simulink model "x1_foc_transform"  (R2024b)
settings: Solver=VariableStepAuto  StartTime=0.0  StopTime=0.5  RelTol=1e-3
undefined symbols (not defined in the file or in its folder): DiscIntNeverNeededParam, Ts
libraries: spspowerguiLib x1
settings Model: Creator=disnox  LastModifiedBy=cd
settings DataIOCC: ReturnWorkspaceOutputs=off
settings DebuggingCC: ParameterPrecisionLossMsg=none
settings RTWCC: GPUComputeCapability=3.5

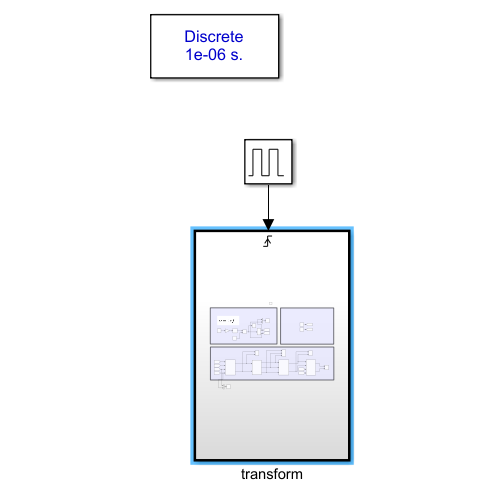
[thumbnail: Simulink's stored preview of the top-level diagram]
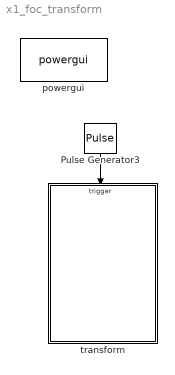
== system x1_foc_transform ==
  Pulse Generator3 : DiscretePulseGenerator  PulseType=Time based  Period=Ts  PulseWidth=50
  powergui : spspowerguiLib/powergui  SimulationMode=Discrete  SampleTime=Ts/100  frequency=60  Iterations=50  frequencyindice=0  Pbase=100e6  ErrMax=1e-4  UnitsV=kV  UnitsW=MW  buscounter=0  FunctionMessages=off  echomessages=off  EnableUseOfTLC=off  CurrentSourceSwitches=off  DisableSnubberDevices=off  DisableRonSwitches=off  DisableVfSwitches=off  DisplayEquations=off  AutomaticDiscreteSolvers=off  SolverType=Tustin/Backward Euler (TBE)  Interpol=off  ExternalGateDelay=off  methode=off  Ts=0  x0status=blocks  SPID=off  SwTol=0  HookPort=off  NonlinearTolerance=1e-4  nMaxIteration=100  ContinueOnMaxIteration=off  RestoreLinks=warning  ResistiveCurrentMeasurement=off  Frange=[0:2:500]  Ylog=off  Xlog=on  ShowGrid=off  save=off  variable=ZData  structure=0  ZoomFFT=off  StartTime=0.0  cycles=1  DisplayStyle=1  fundamental=60  FreqAxis=off  MaxFrequency=1000  frequencyindicesteady=1  RmsSteady=1  display=off
  transform : Subsystem
  wires:
  Pulse Generator3/1 -> transform/Trigger

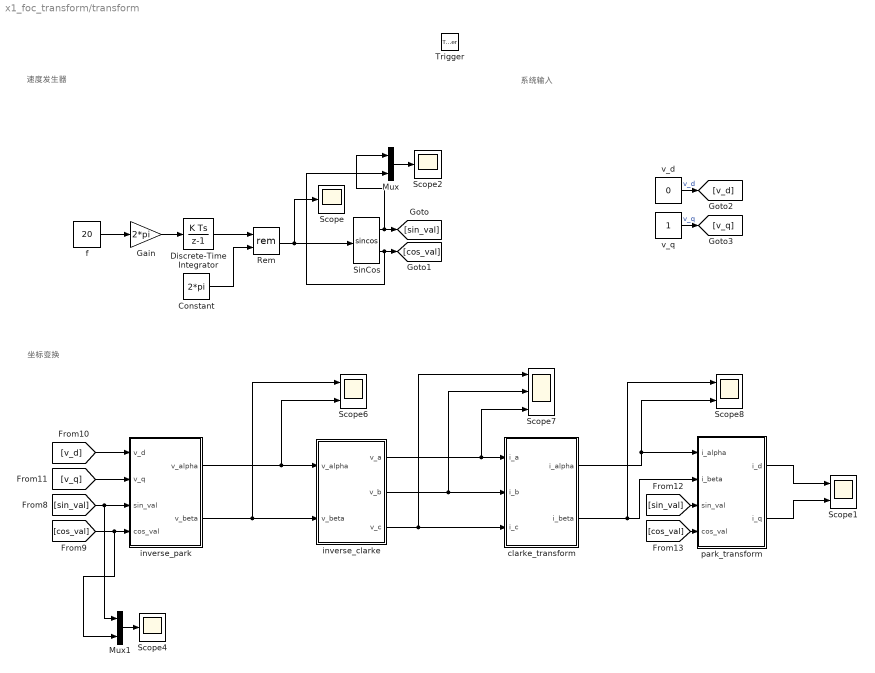
== system x1_foc_transform/transform ==
  note: 系统输入
  note: 速度发生器
  note: 坐标变换
  Trigger : TriggerPort  VariantControl=(inherit)
  Constant : Constant  Value=2*pi
  Discrete-Time Integrator : DiscreteIntegrator  SampleTime=-1  ICPrevOutput=DiscIntNeverNeededParam  ICPrevScaledInput=DiscIntNeverNeededParam
  Gain : Gain  Gain=2*pi
  Mux : Mux  Inputs=2
  Mux1 : Mux  Inputs=2
  Rem : Math  Operator=rem
  Scope : Scope
  Scope1 : Scope  NumInputPorts=2
  Scope2 : Scope
  Scope4 : Scope
  Scope6 : Scope  NumInputPorts=2
  Scope7 : Scope  NumInputPorts=3
  Scope8 : Scope  NumInputPorts=2
  SinCos : Trigonometry  Operator=sincos
  clarke_transform : Subsystem  TreatAsAtomicUnit=on
      settings: RTWSystemCode=Nonreusable function  RTWFcnNameOpts=Use subsystem name
  f : Constant  Value=20
  inverse_clarke : Subsystem  TreatAsAtomicUnit=on
      settings: RTWSystemCode=Nonreusable function  RTWFcnNameOpts=Use subsystem name
  inverse_park : Subsystem  TreatAsAtomicUnit=on
      settings: RTWSystemCode=Nonreusable function  RTWFcnNameOpts=Use subsystem name
  park_transform : Subsystem  TreatAsAtomicUnit=on
      settings: RTWSystemCode=Nonreusable function  RTWFcnNameOpts=Use subsystem name
  v_d : Constant  Value=0
  v_q : Constant
  wires:
  SinCos/1 -> Mux/1, [sin_val]
  SinCos/2 -> Mux/2, [cos_val]
  v_q/1 -> [v_q]  "v_q"
  v_d/1 -> [v_d]  "v_d"
  [cos_val] -> Mux1/2, inverse_park/4(cos_val)
  [sin_val] -> park_transform/3(sin_val)
  [v_d] -> inverse_park/1(v_d)
  [v_q] -> inverse_park/2(v_q)
  [cos_val] -> park_transform/4(cos_val)
  [sin_val] -> Mux1/1, inverse_park/3(sin_val)
  inverse_park/1(v_alpha) -> Scope6/2, inverse_clarke/1(v_alpha)
  clarke_transform/1(i_alpha) -> Scope8/2, park_transform/1(i_alpha)
  clarke_transform/2(i_beta) -> Scope8/1, park_transform/2(i_beta)
  inverse_clarke/1(v_a) -> Scope7/3, clarke_transform/1(i_a)
  inverse_clarke/3(v_c) -> clarke_transform/3(i_c), Scope7/1
  inverse_clarke/2(v_b) -> Scope7/2, clarke_transform/2(i_b)
  inverse_park/2(v_beta) -> Scope6/1, inverse_clarke/2(v_beta)
  park_transform/1(i_d) -> Scope1/1
  park_transform/2(i_q) -> Scope1/2
  Constant/1 -> Rem/2
  f/1 -> Gain/1
  Gain/1 -> Discrete-Time Integrator/1
  Discrete-Time Integrator/1 -> Rem/1
  Rem/1 -> SinCos/1, Scope/1
  Mux/1 -> Scope2/1
  Mux1/1 -> Scope4/1

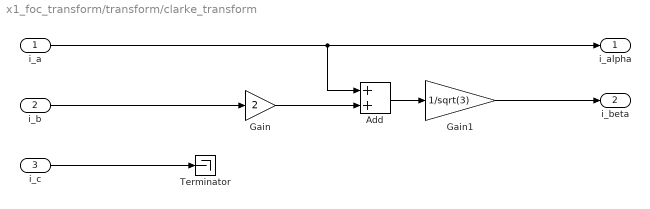
== system x1_foc_transform/transform/clarke_transform ==
  i_a : Inport
  i_b : Inport  Port=2
  i_c : Inport  Port=3
  Add : Sum
  Gain : Gain  Gain=2
  Gain1 : Gain  Gain=1/sqrt(3)
  Terminator : Terminator
  i_alpha : Outport
  i_beta : Outport  Port=2
  wires:
  i_a/1 -> Add/1, i_alpha/1
  i_b/1 -> Gain/1
  Gain/1 -> Add/2
  Add/1 -> Gain1/1
  Gain1/1 -> i_beta/1
  i_c/1 -> Terminator/1

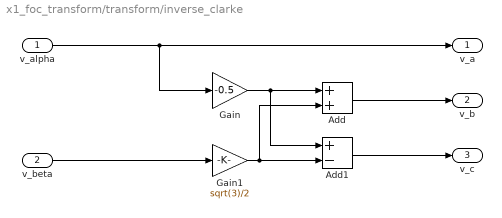
== system x1_foc_transform/transform/inverse_clarke ==
  v_alpha : Inport
  v_beta : Inport  Port=2
  Add : Sum
  Add1 : Sum  Inputs=+-
  Gain : Gain  Gain=-0.5
  Gain1 : Gain  Gain=sqrt(3)/2
  v_a : Outport
  v_b : Outport  Port=2
  v_c : Outport  Port=3
  wires:
  v_alpha/1 -> Gain/1, v_a/1
  Gain/1 -> Add1/1, Add/1
  v_beta/1 -> Gain1/1
  Gain1/1 -> Add/2, Add1/2
  Add/1 -> v_b/1
  Add1/1 -> v_c/1

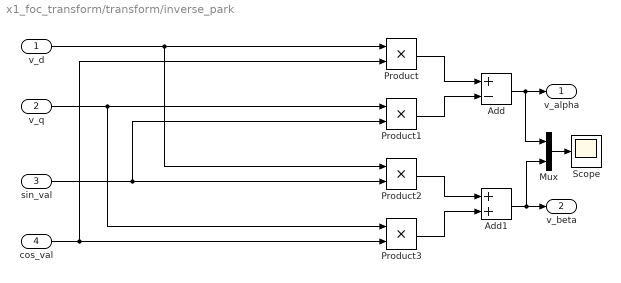
== system x1_foc_transform/transform/inverse_park ==
  v_d : Inport
  v_q : Inport  Port=2
  sin_val : Inport  Port=3
  cos_val : Inport  Port=4
  Add : Sum  Inputs=+-
  Add1 : Sum  AccumDataTypeStr=double
  Mux : Mux  Inputs=2
  Product{,1..3} (4 alike) : Product
  Scope : Scope
  v_alpha : Outport
  v_beta : Outport  Port=2
  wires:
  v_d/1 -> Product2/1, Product/1
  cos_val/1 -> Product3/2, Product/2
  Product/1 -> Add/1
  Product1/1 -> Add/2
  v_q/1 -> Product1/1, Product3/1
  sin_val/1 -> Product2/2, Product1/2
  Add/1 -> Mux/1, v_alpha/1
  Product2/1 -> Add1/1
  Product3/1 -> Add1/2
  Add1/1 -> Mux/2, v_beta/1
  Mux/1 -> Scope/1

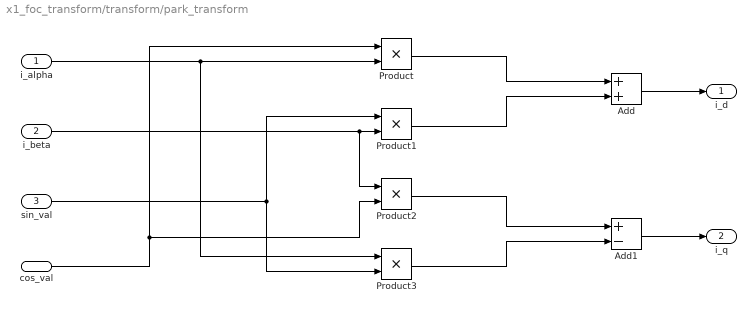
== system x1_foc_transform/transform/park_transform ==
  i_alpha : Inport
  i_beta : Inport  Port=2
  sin_val : Inport  Port=3
  cos_val : Inport  Port=4
  Add : Sum
  Add1 : Sum  Inputs=+-
  Product{,1..3} (4 alike) : Product
  i_d : Outport
  i_q : Outport  Port=2
  wires:
  i_alpha/1 -> Product/2, Product3/1
  cos_val/1 -> Product2/2, Product/1
  sin_val/1 -> Product3/2, Product1/1
  i_beta/1 -> Product2/1, Product1/2
  Product/1 -> Add/1
  Product1/1 -> Add/2
  Add/1 -> i_d/1
  Product2/1 -> Add1/1
  Product3/1 -> Add1/2
  Add1/1 -> i_q/1
